simulink model "arducopter"  (R2021a)
settings: Solver=FixedStepAuto  StartTime=0.0  StopTime=simIn.param.timeEnd  FixedStep=simIn.param.dt  RelTol=1e-3
undefined symbols (not defined in the file or in its folder): DiscIntNeverNeededParam, sim, simIn
libraries: simulink x35, slident x4, vrlib x1
(part 5 of 9)

== system arducopter/Rate Controller/PID Pitch Rate/RAT_FLTD ==
  note: See AP_Math.cpp, calc_lowpass_alpha_dt()
  note: See AC_PID.cpp, update_all()
  note: Alpha Calculation:
      | $\alpha = \frac{\mathrm{d}t}{\mathrm{d}t + 2 \pi f_{\mathrm{Cutoff}}$
  note: Digital Filter:
      | $y_n = (1 - \alpha)y_{n-1} + x \cdot \alpha$
  u : Inport
  cutoff_freq : Inport  Port=2
  ATC input time constant : Constant  Value=simIn.param.dt
  Add : Sum
  Calculate Alpha : Product  Inputs=*/
  Compare To Zero : simulink/Logic and Bit Operations/Compare To Zero  relop=<=  OutDataTypeStr=boolean
  Compare To Zero1 : simulink/Logic and Bit Operations/Compare To Zero  relop=<=  OutDataTypeStr=boolean
  Constant2 : Constant  OutDataTypeStr=single
  Constant3 : Constant  OutDataTypeStr=single
  Constant4 : Constant  OutDataTypeStr=single
  Data Type Conversion1 : DataTypeConversion  OutDataTypeStr=single
  Divide : Product  Inputs=*/
  Gain : Gain  Gain=2*pi
  IC : InitialCondition  Value=simIn.init.PIDP.DerFilt
  Logical Operator : Logic  Operator=OR  AllPortsSameDT=off  OutDataTypeStr=boolean
  Product : Product
  Product1 : Product
  Subtract1 : Sum  Inputs=+-
  Sum : Sum  Inputs=++|
  Switch : Switch  Criteria=u2 > Threshold
  Unit Delay : UnitDelay  SampleTime=-1  HasFrameUpgradeWarning=on
  y : Outport
  wires:
  IC/1 -> y/1, Unit Delay/1
  Sum/1 -> IC/1
  Constant4/1 -> Switch/1
  Logical Operator/1 -> Switch/2
  Compare To Zero1/1 -> Logical Operator/2
  Compare To Zero/1 -> Logical Operator/1
  [cutoff_freq] -> Compare To Zero1/1
  [dt] -> Compare To Zero/1
  [cutoff_freq] -> Gain/1
  ATC input time constant/1 -> Data Type Conversion1/1
  Switch/1 -> [alpha]
  Product/1 -> Sum/1
  Constant3/1 -> Divide/1
  Divide/1 -> Add/2
  u/1 -> Product/2
  cutoff_freq/1 -> [cutoff_freq]
  Gain/1 -> Divide/2
  [dt] -> Calculate Alpha/1, Add/1
  Add/1 -> Calculate Alpha/2
  Calculate Alpha/1 -> Switch/3
  [alpha] -> Product/1
  Constant2/1 -> Subtract1/1
  [alpha] -> Subtract1/2
  Subtract1/1 -> Product1/1
  Unit Delay/1 -> Product1/2
  Product1/1 -> Sum/2
  Data Type Conversion1/1 -> [dt]

== system arducopter/Rate Controller/PID Pitch Rate/RAT_FLTE ==
  note: See AP_Math.cpp, calc_lowpass_alpha_dt()
  note: See AC_PID.cpp, update_all()
  note: Alpha Calculation:
      | $\alpha = \frac{\mathrm{d}t}{\mathrm{d}t + 2 \pi f_{\mathrm{Cutoff}}$
  note: Digital Filter:
      | $y_n = (1 - \alpha)y_{n-1} + x \cdot \alpha$
  u : Inport
  cutoff_freq : Inport  Port=2
  ATC input time constant : Constant  Value=simIn.param.dt
  Add : Sum
  Calculate Alpha : Product  Inputs=*/
  Compare To Zero : simulink/Logic and Bit Operations/Compare To Zero  relop=<=  OutDataTypeStr=boolean
  Compare To Zero1 : simulink/Logic and Bit Operations/Compare To Zero  relop=<=  OutDataTypeStr=boolean
  Constant2 : Constant  OutDataTypeStr=single
  Constant3 : Constant  OutDataTypeStr=single
  Constant4 : Constant  OutDataTypeStr=single
  Data Type Conversion1 : DataTypeConversion  OutDataTypeStr=single
  Divide : Product  Inputs=*/
  Gain : Gain  Gain=2*pi
  IC : InitialCondition  Value=simIn.init.PIDP.ErrFilt
  Logical Operator : Logic  Operator=OR  AllPortsSameDT=off  OutDataTypeStr=boolean
  Product : Product
  Product1 : Product
  Subtract1 : Sum  Inputs=+-
  Sum : Sum  Inputs=++|  OutDataTypeStr=single
  Switch : Switch  Criteria=u2 > Threshold
  Unit Delay : UnitDelay  SampleTime=-1  HasFrameUpgradeWarning=on
  y : Outport
  wires:
  IC/1 -> y/1, Unit Delay/1
  Sum/1 -> IC/1
  Constant4/1 -> Switch/1
  Logical Operator/1 -> Switch/2
  Compare To Zero1/1 -> Logical Operator/2
  Compare To Zero/1 -> Logical Operator/1
  [cutoff_freq] -> Compare To Zero1/1
  [dt] -> Compare To Zero/1
  [cutoff_freq] -> Gain/1
  ATC input time constant/1 -> Data Type Conversion1/1
  Switch/1 -> [alpha]
  Product/1 -> Sum/1
  Constant3/1 -> Divide/1
  Divide/1 -> Add/2
  u/1 -> Product/2
  cutoff_freq/1 -> [cutoff_freq]
  Gain/1 -> Divide/2
  [dt] -> Calculate Alpha/1, Add/1
  Add/1 -> Calculate Alpha/2
  Calculate Alpha/1 -> Switch/3
  [alpha] -> Product/1
  Constant2/1 -> Subtract1/1
  [alpha] -> Subtract1/2
  Subtract1/1 -> Product1/1
  Unit Delay/1 -> Product1/2
  Product1/1 -> Sum/2
  Data Type Conversion1/1 -> [dt]

== system arducopter/Rate Controller/PID Pitch Rate/RAT_FLTT ==
  note: Digital Filter:
      | $y_n = (1 - \alpha)y_{n-1} + x \cdot \alpha$
  note: Alpha Calculation:
      | $\alpha = \frac{\mathrm{d}t}{\mathrm{d}t + 2 \pi f_{\mathrm{Cutoff}}$
  note: See AC_PID.cpp, update_all()
  note: See AP_Math.cpp, calc_lowpass_alpha_dt()
  u : Inport
  cutoff_freq : Inport  Port=2
  ATC input time constant : Constant  Value=simIn.param.dt
  Add : Sum
  Calculate Alpha : Product  Inputs=*/
  Compare To Zero : simulink/Logic and Bit Operations/Compare To Zero  relop=<=  OutDataTypeStr=boolean
  Compare To Zero1 : simulink/Logic and Bit Operations/Compare To Zero  relop=<=  OutDataTypeStr=boolean
  Constant2 : Constant  OutDataTypeStr=single
  Constant3 : Constant  OutDataTypeStr=single
  Constant4 : Constant  OutDataTypeStr=single
  Data Type Conversion1 : DataTypeConversion  OutDataTypeStr=single
  Divide : Product  Inputs=*/
  Gain : Gain  Gain=2*pi
  IC : InitialCondition  Value=simIn.init.PIDP.TarFilt
  Logical Operator : Logic  Operator=OR  AllPortsSameDT=off  OutDataTypeStr=boolean
  Product : Product
  Product1 : Product
  Subtract1 : Sum  Inputs=+-
  Sum : Sum  Inputs=++|
  Switch : Switch  Criteria=u2 > Threshold
  Unit Delay : UnitDelay  SampleTime=-1  HasFrameUpgradeWarning=on
  y : Outport
  wires:
  IC/1 -> Unit Delay/1, y/1
  Unit Delay/1 -> Product1/2
  Sum/1 -> IC/1
  Product1/1 -> Sum/2
  Subtract1/1 -> Product1/1
  [alpha] -> Subtract1/2
  Constant2/1 -> Subtract1/1
  [alpha] -> Product/1
  Calculate Alpha/1 -> Switch/3
  Add/1 -> Calculate Alpha/2
  [dt] -> Add/1, Calculate Alpha/1
  Gain/1 -> Divide/2
  cutoff_freq/1 -> [cutoff_freq]
  u/1 -> Product/2
  Divide/1 -> Add/2
  Constant3/1 -> Divide/1
  Product/1 -> Sum/1
  Switch/1 -> [alpha]
  ATC input time constant/1 -> Data Type Conversion1/1
  [cutoff_freq] -> Gain/1
  [dt] -> Compare To Zero/1
  [cutoff_freq] -> Compare To Zero1/1
  Compare To Zero/1 -> Logical Operator/1
  Compare To Zero1/1 -> Logical Operator/2
  Logical Operator/1 -> Switch/2
  Constant4/1 -> Switch/1
  Data Type Conversion1/1 -> [dt]

== system arducopter/Rate Controller/PID Pitch Rate/Slew Limiter ==
  note: Data Store Memory Elements: Global variables of subsystem
  note: Slew Limiter
      |
      | Calculates the slew limit modifiert Dmod for the P and D part of the controller. The calculation of Dmod is taken from SlewLimiter::modifier() in SlewLimiter.cpp.
  p_out : Inport
  sr_max : Inport  Port=2
  sr_tau : Inport  Port=3
  sr_flt_f : Inport  Port=4
  clock : Inport  Port=5
  d_out : Inport  Port=6
  ATC sample time1 : Constant  Value=simIn.param.dt
  Calculate Dmod1 : MATLAB Function  TreatAsAtomicUnit=on  SystemSampleTime=0.0025
  Constant7 : Constant  Value=simIn.param.LOOP_RATE
  Data Store Memory : DataStoreMemory  DataStoreName=pos_event_stored  ReadBeforeWriteMsg=warning  WriteAfterWriteMsg=warning  WriteAfterReadMsg=warning  InitialValue=false  ShowAdditionalParam=off  OutDataTypeStr=boolean
  Data Store Memory1 : DataStoreMemory  DataStoreName=neg_event_stored  ReadBeforeWriteMsg=warning  WriteAfterWriteMsg=warning  WriteAfterReadMsg=warning  InitialValue=false  ShowAdditionalParam=off  OutDataTypeStr=boolean
  Data Store Memory10 : DataStoreMemory  DataStoreName=modifier_slew_rate  ReadBeforeWriteMsg=warning  WriteAfterWriteMsg=warning  WriteAfterReadMsg=warning  InitialValue=simIn.init.PIDP.SrOut  ShowAdditionalParam=off  OutDataTypeStr=single
  Data Store Memory11 : DataStoreMemory  DataStoreName=output_slew_rate  ReadBeforeWriteMsg=warning  WriteAfterWriteMsg=warning  WriteAfterReadMsg=warning  InitialValue=simIn.init.PIDP.SrOut  ShowAdditionalParam=off  OutDataTypeStr=single
  Data Store Memory2 : DataStoreMemory  DataStoreName=pos_event_idx  ReadBeforeWriteMsg=warning  WriteAfterWriteMsg=warning  WriteAfterReadMsg=warning  InitialValue=1  ShowAdditionalParam=off  OutDataTypeStr=int8
  Data Store Memory3 : DataStoreMemory  DataStoreName=neg_event_idx  ReadBeforeWriteMsg=warning  WriteAfterWriteMsg=warning  WriteAfterReadMsg=warning  InitialValue=1  ShowAdditionalParam=off  OutDataTypeStr=int8
  Data Store Memory4 : DataStoreMemory  DataStoreName=pos_event_ms  ReadBeforeWriteMsg=warning  WriteAfterWriteMsg=warning  WriteAfterReadMsg=warning  InitialValue=[0 0]  ShowAdditionalParam=off  OutDataTypeStr=uint32  Dimensions=2
  Data Store Memory5 : DataStoreMemory  DataStoreName=neg_event_ms  ReadBeforeWriteMsg=warning  WriteAfterWriteMsg=warning  WriteAfterReadMsg=warning  InitialValue=[0 0]  ShowAdditionalParam=off  OutDataTypeStr=uint32  Dimensions=2
  Data Store Memory6 : DataStoreMemory  DataStoreName=max_pos_slew_rate  ReadBeforeWriteMsg=warning  WriteAfterWriteMsg=warning  WriteAfterReadMsg=warning  ShowAdditionalParam=off  OutDataTypeStr=single
  Data Store Memory7 : DataStoreMemory  DataStoreName=max_pos_slew_event_ms  ReadBeforeWriteMsg=warning  WriteAfterWriteMsg=warning  WriteAfterReadMsg=warning  ShowAdditionalParam=off  OutDataTypeStr=uint32
  Data Store Memory8 : DataStoreMemory  DataStoreName=max_neg_slew_rate  ReadBeforeWriteMsg=warning  WriteAfterWriteMsg=warning  WriteAfterReadMsg=warning  ShowAdditionalParam=off  OutDataTypeStr=single
  Data Store Memory9 : DataStoreMemory  DataStoreName=max_neg_slew_event_ms  ReadBeforeWriteMsg=warning  WriteAfterWriteMsg=warning  WriteAfterReadMsg=warning  ShowAdditionalParam=off  OutDataTypeStr=uint32
  Data Store Read : DataStoreRead  DataStoreName=modifier_slew_rate  DataStoreElements=modifier_slew_rate  IndexOptions=Index vector (dialog)  Indices=1  OutputSizes=1
  Data Store Read1 : DataStoreRead  DataStoreName=output_slew_rate  DataStoreElements=output_slew_rate  IndexOptions=Index vector (dialog)  Indices=1  OutputSizes=1
  Data Type Conversion1 : DataTypeConversion  OutDataTypeStr=single
  IC : InitialCondition  Value=2*simIn.init.PIDP.SrOut
  Lowpass Filter1 : MATLAB Function  TreatAsAtomicUnit=on
  Subsystem : Subsystem
  Terminator : Terminator
  Terminator1 : Terminator
  Unit Delay1 : UnitDelay  SampleTime=-1  HasFrameUpgradeWarning=on
  Dmod : Outport
  wires:
  Constant7/1 -> Lowpass Filter1/3(loop_rate)
  sr_flt_f/1 -> Lowpass Filter1/2(cutoff_freq)
  Lowpass Filter1/1(out) -> IC/1  "pitchRateSrFilt"
  Unit Delay1/1 -> Lowpass Filter1/4(out_last)
  Calculate Dmod1/1(Dmod) -> Dmod/1  "pitchRateDmod"
  sr_max/1 -> Calculate Dmod1/2(sr_max)
  sr_tau/1 -> Calculate Dmod1/3(sr_tau)
  ATC sample time1/1 -> Data Type Conversion1/1
  Data Store Read/1 -> Terminator/1  "pitchRateSrMod"
  Data Store Read1/1 -> Terminator1/1  "pitchRateSrOut"
  p_out/1 -> Subsystem/1(p_out)
  d_out/1 -> Subsystem/2(d_out)
  Subsystem/1(sr_raw) -> Lowpass Filter1/1(in)  "pitchRateSrRaw"
  Data Type Conversion1/1 -> Calculate Dmod1/4(dt)
  IC/1 -> Calculate Dmod1/1(slew_rate), Unit Delay1/1
  clock/1 -> Calculate Dmod1/5(time)

== system arducopter/Rate Controller/PID Roll Rate/Calc Derivative ==
  e : Inport
  ATC input time constant : Constant  Value=simIn.param.dt
  Data Type Conversion : DataTypeConversion  OutDataTypeStr=single
  Divide : Product  Inputs=*/
  Sum : Sum  Inputs=|+-
  Unit Delay : UnitDelay  SampleTime=-1  HasFrameUpgradeWarning=on
  derivative : Outport
  wires:
  e/1 -> Sum/1, Unit Delay/1
  Unit Delay/1 -> Sum/2
  Sum/1 -> Divide/1
  ATC input time constant/1 -> Data Type Conversion/1
  Divide/1 -> derivative/1
  Data Type Conversion/1 -> Divide/2

== system arducopter/Rate Controller/PID Roll Rate/I ==
  note: Integrator, see AC_PID::update_i()
  e : Inport
  limit_flg : Inport  Port=2
  ki : Inport  Port=3
  i_max : Inport  Port=4
  Constant1 : Constant  Value=simIn.param.dt
  Data Type Conversion : DataTypeConversion  OutDataTypeStr=single
  IC1 : InitialCondition  Value=simIn.init.PIDR.I
  Integrator : MATLAB Function  TreatAsAtomicUnit=on
  Unit Delay1 : UnitDelay  SampleTime=-1  HasFrameUpgradeWarning=on
  integrator : Outport
  wires:
  [integrator_out] -> integrator/1
  Constant1/1 -> Data Type Conversion/1
  limit_flg/1 -> Integrator/3(limit_flg)
  [integrator_out] -> Unit Delay1/1
  IC1/1 -> [integrator_out]
  Unit Delay1/1 -> Integrator/2(integrator)
  ki/1 -> Integrator/4(ki)
  i_max/1 -> Integrator/5(i_max)
  e/1 -> Integrator/1(error)
  Integrator/1(integrator_out) -> IC1/1
  Data Type Conversion/1 -> Integrator/6(dt)

== system arducopter/Rate Controller/PID Roll Rate/RAT_FLTD ==
  note: Digital Filter:
      | $y_n = (1 - \alpha)y_{n-1} + x \cdot \alpha$
  note: Alpha Calculation:
      | $\alpha = \frac{\mathrm{d}t}{\mathrm{d}t + 2 \pi T_{\mathrm{Cutoff}}$
  note: See AC_PID.cpp, update_all()
  note: See AP_Math.cpp, calc_lowpass_alpha_dt()
  u : Inport
  cutoff_freq : Inport  Port=2
  ATC input time constant : Constant  Value=simIn.param.dt
  Add : Sum
  Calculate Alpha : Product  Inputs=*/
  Compare To Zero : simulink/Logic and Bit Operations/Compare To Zero  relop=<=  OutDataTypeStr=boolean
  Compare To Zero1 : simulink/Logic and Bit Operations/Compare To Zero  relop=<=  OutDataTypeStr=boolean
  Constant : Constant  Commented=on
  Constant1 : Constant  Commented=on
  Constant2 : Constant  OutDataTypeStr=single
  Constant3 : Constant  OutDataTypeStr=single
  Constant4 : Constant  OutDataTypeStr=single
  Data Type Conversion : DataTypeConversion  OutDataTypeStr=single
  Discrete Filter : DiscreteFilter  Commented=on  NumeratorSource=Input port  DenominatorSource=Input port  a0EqualsOne=on
      settings: InputPortMap=u0,p1,p3
  Divide : Product  Inputs=*/
  From : From  Commented=on  GotoTag=alpha
  From1 : From  Commented=on  GotoTag=alpha
  Gain : Gain  Gain=2*pi
  Gain1 : Gain  Commented=on  Gain=-1
  IC : InitialCondition  Value=simIn.init.PIDR.DerFilt
  Logical Operator : Logic  Operator=OR  AllPortsSameDT=off  OutDataTypeStr=boolean
  Product : Product
  Product1 : Product
  Subtract : Sum  Commented=on  Inputs=+-
  Subtract1 : Sum  Inputs=+-
  Sum : Sum  Inputs=++|  AccumDataTypeStr=single
  Switch : Switch  Criteria=u2 > Threshold
  Unit Delay : UnitDelay  SampleTime=-1  HasFrameUpgradeWarning=on
  Vector Concatenate : Concatenate  Commented=on
  degree2radian1 : Gain  Commented=on  Gain=pi/180
  y : Outport
  wires:
  Product1/1 -> Sum/2
  Unit Delay/1 -> Product1/2
  Subtract1/1 -> Product1/1
  [alpha] -> Subtract1/2
  Constant2/1 -> Subtract1/1
  [alpha] -> Product/1
  Vector Concatenate/1 -> Discrete Filter/3
  Constant1/1 -> Vector Concatenate/1
  Gain1/1 -> Vector Concatenate/2
  Subtract/1 -> Gain1/1
  Constant/1 -> Subtract/1
  From1/1 -> Subtract/2
  From/1 -> Discrete Filter/2
  Calculate Alpha/1 -> Switch/3
  Add/1 -> Calculate Alpha/2
  [dt] -> Add/1, Calculate Alpha/1
  Gain/1 -> Divide/2
  cutoff_freq/1 -> [cutoff_freq]
  Discrete Filter/1 -> degree2radian1/1
  u/1 -> Product/2
  Divide/1 -> Add/2
  Constant3/1 -> Divide/1
  Product/1 -> Sum/1
  Switch/1 -> [alpha]
  ATC input time constant/1 -> Data Type Conversion/1
  [cutoff_freq] -> Gain/1
  [dt] -> Compare To Zero/1
  [cutoff_freq] -> Compare To Zero1/1
  Compare To Zero/1 -> Logical Operator/1
  Compare To Zero1/1 -> Logical Operator/2
  Logical Operator/1 -> Switch/2
  Constant4/1 -> Switch/1
  Sum/1 -> IC/1
  IC/1 -> Unit Delay/1, y/1
  Data Type Conversion/1 -> [dt]

== system arducopter/Rate Controller/PID Roll Rate/RAT_FLTE ==
  note: Digital Filter:
      | $y_n = (1 - \alpha)y_{n-1} + x \cdot \alpha$
  note: Alpha Calculation:
      | $\alpha = \frac{\mathrm{d}t}{\mathrm{d}t + 2 \pi f_{\mathrm{Cutoff}}$
  note: See AC_PID.cpp, update_all()
  note: See AP_Math.cpp, calc_lowpass_alpha_dt()
  u : Inport
  cutoff_freq : Inport  Port=2
  ATC input time constant : Constant  Value=simIn.param.dt
  Add : Sum
  Calculate Alpha : Product  Inputs=*/
  Compare To Zero : simulink/Logic and Bit Operations/Compare To Zero  relop=<=  OutDataTypeStr=boolean
  Compare To Zero1 : simulink/Logic and Bit Operations/Compare To Zero  relop=<=  OutDataTypeStr=boolean
  Constant2 : Constant  OutDataTypeStr=single
  Constant3 : Constant  OutDataTypeStr=single
  Constant4 : Constant  OutDataTypeStr=single
  Data Type Conversion : DataTypeConversion  OutDataTypeStr=single
  Divide : Product  Inputs=*/
  Gain : Gain  Gain=2*pi
  IC : InitialCondition  Value=simIn.init.PIDR.ErrFilt
  Logical Operator : Logic  Operator=OR  AllPortsSameDT=off  OutDataTypeStr=boolean
  Product : Product
  Product1 : Product
  Subtract1 : Sum  Inputs=+-
  Sum : Sum  Inputs=++|  OutDataTypeStr=single
  Switch : Switch  Criteria=u2 > Threshold
  Unit Delay : UnitDelay  SampleTime=-1  HasFrameUpgradeWarning=on
  y : Outport
  wires:
  Product1/1 -> Sum/2
  Unit Delay/1 -> Product1/2
  Subtract1/1 -> Product1/1
  [alpha] -> Subtract1/2
  Constant2/1 -> Subtract1/1
  [alpha] -> Product/1
  Calculate Alpha/1 -> Switch/3
  Add/1 -> Calculate Alpha/2
  [dt] -> Add/1, Calculate Alpha/1
  Gain/1 -> Divide/2
  cutoff_freq/1 -> [cutoff_freq]
  u/1 -> Product/2
  Divide/1 -> Add/2
  Constant3/1 -> Divide/1
  Product/1 -> Sum/1
  Switch/1 -> [alpha]
  ATC input time constant/1 -> Data Type Conversion/1
  [cutoff_freq] -> Gain/1
  [dt] -> Compare To Zero/1
  [cutoff_freq] -> Compare To Zero1/1
  Compare To Zero/1 -> Logical Operator/1
  Compare To Zero1/1 -> Logical Operator/2
  Logical Operator/1 -> Switch/2
  Constant4/1 -> Switch/1
  Sum/1 -> IC/1
  IC/1 -> Unit Delay/1, y/1
  Data Type Conversion/1 -> [dt]

== system arducopter/Rate Controller/PID Roll Rate/RAT_FLTT ==
  note: See AP_Math.cpp, calc_lowpass_alpha_dt()
  note: See AC_PID.cpp, update_all()
  note: Alpha Calculation:
      | $\alpha = \frac{\mathrm{d}t}{\mathrm{d}t + 2 \pi f_{\mathrm{Cutoff}}$
  note: Digital Filter:
      | $y_n = (1 - \alpha)y_{n-1} + x \cdot \alpha$
  u : Inport
  cutoff_freq : Inport  Port=2
  ATC input time constant : Constant  Value=simIn.param.dt
  Add : Sum
  Calculate Alpha : Product  Inputs=*/
  Compare To Zero : simulink/Logic and Bit Operations/Compare To Zero  relop=<=  OutDataTypeStr=boolean
  Compare To Zero1 : simulink/Logic and Bit Operations/Compare To Zero  relop=<=  OutDataTypeStr=boolean
  Constant2 : Constant  OutDataTypeStr=single
  Constant3 : Constant  OutDataTypeStr=single
  Constant4 : Constant  OutDataTypeStr=single
  Data Type Conversion : DataTypeConversion  OutDataTypeStr=single
  Divide : Product  Inputs=*/
  Gain : Gain  Gain=2*pi
  IC : InitialCondition  Value=simIn.init.PIDR.TarFilt
  Logical Operator : Logic  Operator=OR  AllPortsSameDT=off  OutDataTypeStr=boolean
  Product : Product
  Product1 : Product
  Subtract1 : Sum  Inputs=+-
  Sum : Sum  Inputs=++|
  Switch : Switch  Criteria=u2 > Threshold
  Unit Delay : UnitDelay  SampleTime=-1  HasFrameUpgradeWarning=on
  y : Outport
  wires:
  Constant4/1 -> Switch/1
  Logical Operator/1 -> Switch/2
  Compare To Zero1/1 -> Logical Operator/2
  Compare To Zero/1 -> Logical Operator/1
  [cutoff_freq] -> Compare To Zero1/1
  [dt] -> Compare To Zero/1
  [cutoff_freq] -> Gain/1
  ATC input time constant/1 -> Data Type Conversion/1
  Switch/1 -> [alpha]
  Product/1 -> Sum/1
  Constant3/1 -> Divide/1
  Divide/1 -> Add/2
  u/1 -> Product/2
  cutoff_freq/1 -> [cutoff_freq]
  Gain/1 -> Divide/2
  [dt] -> Calculate Alpha/1, Add/1
  Add/1 -> Calculate Alpha/2
  Calculate Alpha/1 -> Switch/3
  [alpha] -> Product/1
  Constant2/1 -> Subtract1/1
  [alpha] -> Subtract1/2
  Subtract1/1 -> Product1/1
  Product1/1 -> Sum/2
  Sum/1 -> IC/1
  Unit Delay/1 -> Product1/2
  IC/1 -> y/1, Unit Delay/1
  Data Type Conversion/1 -> [dt]

== system arducopter/Rate Controller/PID Roll Rate/Slew Limiter ==
  note: Data Store Memory Elements: Global variables of subsystem
  note: Slew Limiter
      |
      | Calculates the slew limit modifiert Dmod for the P and D part of the controller. The calculation of Dmod is taken from SlewLimiter::modifier() in SlewLimiter.cpp.
  p_out : Inport
  sr_max : Inport  Port=2
  sr_tau : Inport  Port=3
  sr_flt_f : Inport  Port=4
  clock : Inport  Port=5
  d_out : Inport  Port=6
  Calculate Dmod : MATLAB Function  TreatAsAtomicUnit=on  SystemSampleTime=0.0025
  Constant7 : Constant  Value=simIn.param.LOOP_RATE
  Data Store Memory : DataStoreMemory  DataStoreName=pos_event_stored  ReadBeforeWriteMsg=warning  WriteAfterWriteMsg=warning  WriteAfterReadMsg=warning  InitialValue=false  ShowAdditionalParam=off  OutDataTypeStr=boolean
  Data Store Memory1 : DataStoreMemory  DataStoreName=neg_event_stored  ReadBeforeWriteMsg=warning  WriteAfterWriteMsg=warning  WriteAfterReadMsg=warning  InitialValue=false  ShowAdditionalParam=off  OutDataTypeStr=boolean
  Data Store Memory10 : DataStoreMemory  DataStoreName=modifier_slew_rate  ReadBeforeWriteMsg=warning  WriteAfterWriteMsg=warning  WriteAfterReadMsg=warning  InitialValue=simIn.init.PIDR.SROut  ShowAdditionalParam=off  OutDataTypeStr=single
  Data Store Memory11 : DataStoreMemory  DataStoreName=output_slew_rate  ReadBeforeWriteMsg=warning  WriteAfterWriteMsg=warning  WriteAfterReadMsg=warning  InitialValue=simIn.init.PIDR.SROut  ShowAdditionalParam=off  OutDataTypeStr=single
  Data Store Memory2 : DataStoreMemory  DataStoreName=pos_event_idx  ReadBeforeWriteMsg=warning  WriteAfterWriteMsg=warning  WriteAfterReadMsg=warning  InitialValue=1  ShowAdditionalParam=off  OutDataTypeStr=int8
  Data Store Memory3 : DataStoreMemory  DataStoreName=neg_event_idx  ReadBeforeWriteMsg=warning  WriteAfterWriteMsg=warning  WriteAfterReadMsg=warning  InitialValue=1  ShowAdditionalParam=off  OutDataTypeStr=int8
  Data Store Memory4 : DataStoreMemory  DataStoreName=pos_event_ms  ReadBeforeWriteMsg=warning  WriteAfterWriteMsg=warning  WriteAfterReadMsg=warning  InitialValue=[0 0]  ShowAdditionalParam=off  OutDataTypeStr=uint32  Dimensions=2
  Data Store Memory5 : DataStoreMemory  DataStoreName=neg_event_ms  ReadBeforeWriteMsg=warning  WriteAfterWriteMsg=warning  WriteAfterReadMsg=warning  InitialValue=[0 0]  ShowAdditionalParam=off  OutDataTypeStr=uint32  Dimensions=2
  Data Store Memory6 : DataStoreMemory  DataStoreName=max_pos_slew_rate  ReadBeforeWriteMsg=warning  WriteAfterWriteMsg=warning  WriteAfterReadMsg=warning  ShowAdditionalParam=off  OutDataTypeStr=single
  Data Store Memory7 : DataStoreMemory  DataStoreName=max_pos_slew_event_ms  ReadBeforeWriteMsg=warning  WriteAfterWriteMsg=warning  WriteAfterReadMsg=warning  ShowAdditionalParam=off  OutDataTypeStr=uint32
  Data Store Memory8 : DataStoreMemory  DataStoreName=max_neg_slew_rate  ReadBeforeWriteMsg=warning  WriteAfterWriteMsg=warning  WriteAfterReadMsg=warning  ShowAdditionalParam=off  OutDataTypeStr=single
  Data Store Memory9 : DataStoreMemory  DataStoreName=max_neg_slew_event_ms  ReadBeforeWriteMsg=warning  WriteAfterWriteMsg=warning  WriteAfterReadMsg=warning  ShowAdditionalParam=off  OutDataTypeStr=uint32
  Data Store Read : DataStoreRead  DataStoreName=modifier_slew_rate  DataStoreElements=modifier_slew_rate  IndexOptions=Index vector (dialog)  Indices=1  OutputSizes=1
  Data Store Read1 : DataStoreRead  DataStoreName=output_slew_rate  DataStoreElements=output_slew_rate  IndexOptions=Index vector (dialog)  Indices=1  OutputSizes=1
  Data Type Conversion1 : DataTypeConversion  OutDataTypeStr=single
  IC : InitialCondition  Value=2*simIn.init.PIDR.SROut
  Lowpass Filter : MATLAB Function  TreatAsAtomicUnit=on
  Sample time : Constant  Value=simIn.param.dt
  Subsystem : Subsystem
  Terminator : Terminator
  Terminator1 : Terminator
  Unit Delay1 : UnitDelay  SampleTime=-1  HasFrameUpgradeWarning=on
  Dmod : Outport
  wires:
  Constant7/1 -> Lowpass Filter/3(loop_rate)
  sr_flt_f/1 -> Lowpass Filter/2(cutoff_freq)
  Lowpass Filter/1(out) -> IC/1  "rollRateSrFilt"
  Unit Delay1/1 -> Lowpass Filter/4(out_last)
  Calculate Dmod/1(Dmod) -> Dmod/1  "rollRateDmod"
  sr_max/1 -> Calculate Dmod/2(sr_max)
  sr_tau/1 -> Calculate Dmod/3(sr_tau)
  Sample time/1 -> Data Type Conversion1/1
  Data Store Read/1 -> Terminator/1  "rollRateSrModifier"
  Data Store Read1/1 -> Terminator1/1  "rollRateSrOut"
  p_out/1 -> Subsystem/1(p_out)
  d_out/1 -> Subsystem/2(d_out)
  Subsystem/1(sr_raw) -> Lowpass Filter/1(in)  "rollRateSrRaw"
  Data Type Conversion1/1 -> Calculate Dmod/4(dt)
  IC/1 -> Calculate Dmod/1(slew_rate), Unit Delay1/1
  clock/1 -> Calculate Dmod/5(time)

== system arducopter/Rate Controller/PID Yaw Rate/Calc Derivative ==
  e : Inport
  ATC input time constant : Constant  Value=simIn.param.dt
  Divide : Product  Inputs=*/
  Sum : Sum  Inputs=|+-
  Unit Delay : UnitDelay  SampleTime=-1  HasFrameUpgradeWarning=on
  derivative : Outport
  wires:
  e/1 -> Sum/1, Unit Delay/1
  Unit Delay/1 -> Sum/2
  Sum/1 -> Divide/1
  ATC input time constant/1 -> Divide/2
  Divide/1 -> derivative/1

== system arducopter/Rate Controller/PID Yaw Rate/I ==
  note: Integrator, see AC_PID::update_i()
  e : Inport
  limit_flg : Inport  Port=2
  ki : Inport  Port=3
  i_max : Inport  Port=4
  Constant1 : Constant  Value=simIn.param.dt
  Data Type Conversion1 : DataTypeConversion  OutDataTypeStr=single
  IC1 : InitialCondition  Value=simIn.init.PIDY.I
  Integrator : MATLAB Function  TreatAsAtomicUnit=on
  Unit Delay1 : UnitDelay  InitialCondition=single(0)  SampleTime=-1  HasFrameUpgradeWarning=on
  integrator : Outport
  wires:
  e/1 -> Integrator/1(error)
  Integrator/1(integrator_out) -> IC1/1
  [integrator_out] -> integrator/1
  Constant1/1 -> Data Type Conversion1/1
  limit_flg/1 -> Integrator/3(limit_flg)
  [integrator_out] -> Unit Delay1/1
  IC1/1 -> [integrator_out]
  Unit Delay1/1 -> Integrator/2(integrator)
  ki/1 -> Integrator/4(ki)
  i_max/1 -> Integrator/5(i_max)
  Data Type Conversion1/1 -> Integrator/6(dt)

== system arducopter/Rate Controller/PID Yaw Rate/RAT_FLTD ==
  note: Digital Filter:
      | $y_n = (1 - \alpha)y_{n-1} + x \cdot \alpha$
  note: Alpha Calculation:
      | $\alpha = \frac{\mathrm{d}t}{\mathrm{d}t + 2 \pi f_{\mathrm{Cutoff}}$
  note: See AC_PID.cpp, update_all()
  note: See AP_Math.cpp, line 393.
  u : Inport
  cutoff_freq : Inport  Port=2
  ATC input time constant : Constant  Value=simIn.param.dt
  Add : Sum
  Calculate Alpha : Product  Inputs=*/
  Compare To Zero : simulink/Logic and Bit Operations/Compare To Zero  relop=<=  OutDataTypeStr=boolean
  Compare To Zero1 : simulink/Logic and Bit Operations/Compare To Zero  relop=<=  OutDataTypeStr=boolean
  Constant2 : Constant  OutDataTypeStr=single
  Constant3 : Constant  OutDataTypeStr=single
  Constant4 : Constant  OutDataTypeStr=single
  Data Type Conversion1 : DataTypeConversion  OutDataTypeStr=single
  Divide : Product  Inputs=*/
  Gain : Gain  Gain=2*pi
  IC : InitialCondition  Value=simIn.init.PIDY.DerFilt
  Logical Operator : Logic  Operator=OR  AllPortsSameDT=off  OutDataTypeStr=boolean
  Product : Product
  Product1 : Product
  Subtract1 : Sum  Inputs=+-
  Sum : Sum  Inputs=++|  OutDataTypeStr=single
  Switch : Switch  Criteria=u2 > Threshold
  Unit Delay : UnitDelay  SampleTime=-1  HasFrameUpgradeWarning=on
  y : Outport
  wires:
  Product1/1 -> Sum/2
  Unit Delay/1 -> Product1/2
  Subtract1/1 -> Product1/1
  [alpha] -> Subtract1/2
  Constant2/1 -> Subtract1/1
  [alpha] -> Product/1
  Calculate Alpha/1 -> Switch/3
  Add/1 -> Calculate Alpha/2
  [dt] -> Add/1, Calculate Alpha/1
  Gain/1 -> Divide/2
  cutoff_freq/1 -> [cutoff_freq]
  u/1 -> Product/2
  Divide/1 -> Add/2
  Constant3/1 -> Divide/1
  Product/1 -> Sum/1
  Switch/1 -> [alpha]
  ATC input time constant/1 -> Data Type Conversion1/1
  [cutoff_freq] -> Gain/1
  [dt] -> Compare To Zero/1
  [cutoff_freq] -> Compare To Zero1/1
  Compare To Zero/1 -> Logical Operator/1
  Compare To Zero1/1 -> Logical Operator/2
  Logical Operator/1 -> Switch/2
  Constant4/1 -> Switch/1
  Sum/1 -> IC/1
  IC/1 -> Unit Delay/1, y/1
  Data Type Conversion1/1 -> [dt]

== system arducopter/Rate Controller/PID Yaw Rate/RAT_FLTE ==
  note: Digital Filter:
      | $y_n = (1 - \alpha)y_{n-1} + x \cdot \alpha$
  note: Alpha Calculation:
      | $\alpha = \frac{\mathrm{d}t}{\mathrm{d}t + 2 \pi f_{\mathrm{Cutoff}}$
  note: See AC_PID.cpp, update_all()
  note: See AP_Math.cpp, line 393.
  u : Inport
  cutoff_freq : Inport  Port=2
  ATC input time constant : Constant  Value=simIn.param.dt
  Add : Sum
  Calculate Alpha : Product  Inputs=*/
  Compare To Zero : simulink/Logic and Bit Operations/Compare To Zero  relop=<=  OutDataTypeStr=boolean
  Compare To Zero1 : simulink/Logic and Bit Operations/Compare To Zero  relop=<=  OutDataTypeStr=boolean
  Constant : Constant  Commented=on
  Constant1 : Constant  Commented=on
  Constant2 : Constant  OutDataTypeStr=single
  Constant3 : Constant  OutDataTypeStr=single
  Constant4 : Constant  OutDataTypeStr=single
  Data Type Conversion1 : DataTypeConversion  OutDataTypeStr=single
  Discrete Filter : DiscreteFilter  Commented=on  NumeratorSource=Input port  DenominatorSource=Input port  a0EqualsOne=on
      settings: InputPortMap=u0,p1,p3
  Divide : Product  Inputs=*/
  From : From  Commented=on  GotoTag=alpha
  From1 : From  Commented=on  GotoTag=alpha
  Gain : Gain  Gain=2*pi
  Gain1 : Gain  Commented=on  Gain=-1
  IC : InitialCondition  Value=simIn.init.PIDY.ErrFilt
  Logical Operator : Logic  Operator=OR  AllPortsSameDT=off  OutDataTypeStr=boolean
  Product : Product
  Product1 : Product
  Subtract : Sum  Commented=on  Inputs=+-
  Subtract1 : Sum  Inputs=+-
  Sum : Sum  Inputs=++|  OutDataTypeStr=single
  Switch : Switch  Criteria=u2 > Threshold
  Unit Delay : UnitDelay  SampleTime=-1  HasFrameUpgradeWarning=on
  Vector Concatenate : Concatenate  Commented=on
  degree2radian1 : Gain  Commented=on  Gain=pi/180
  y : Outport
  wires:
  Product1/1 -> Sum/2
  Unit Delay/1 -> Product1/2
  Subtract1/1 -> Product1/1
  [alpha] -> Subtract1/2
  Constant2/1 -> Subtract1/1
  [alpha] -> Product/1
  Vector Concatenate/1 -> Discrete Filter/3
  Constant1/1 -> Vector Concatenate/1
  Gain1/1 -> Vector Concatenate/2
  Subtract/1 -> Gain1/1
  Constant/1 -> Subtract/1
  From1/1 -> Subtract/2
  From/1 -> Discrete Filter/2
  Calculate Alpha/1 -> Switch/3
  Add/1 -> Calculate Alpha/2
  [dt] -> Add/1, Calculate Alpha/1
  Gain/1 -> Divide/2
  cutoff_freq/1 -> [cutoff_freq]
  Discrete Filter/1 -> degree2radian1/1
  u/1 -> Product/2
  Divide/1 -> Add/2
  Constant3/1 -> Divide/1
  Product/1 -> Sum/1
  Switch/1 -> [alpha]
  ATC input time constant/1 -> Data Type Conversion1/1
  [cutoff_freq] -> Gain/1
  [dt] -> Compare To Zero/1
  [cutoff_freq] -> Compare To Zero1/1
  Compare To Zero/1 -> Logical Operator/1
  Compare To Zero1/1 -> Logical Operator/2
  Logical Operator/1 -> Switch/2
  Constant4/1 -> Switch/1
  Sum/1 -> IC/1
  IC/1 -> Unit Delay/1, y/1
  Data Type Conversion1/1 -> [dt]

== system arducopter/Rate Controller/PID Yaw Rate/RAT_FLTT ==
  note: See AP_Math.cpp, line 393.
  note: See AC_PID.cpp, update_all()
  note: Alpha Calculation:
      | $\alpha = \frac{\mathrm{d}t}{\mathrm{d}t + 2 \pi f_{\mathrm{Cutoff}}$
  note: Digital Filter:
      | $y_n = (1 - \alpha)y_{n-1} + x \cdot \alpha$
  u : Inport
  cutoff_freq : Inport  Port=2
  ATC input time constant : Constant  Value=simIn.param.dt
  Add : Sum
  Calculate Alpha : Product  Inputs=*/
  Compare To Zero : simulink/Logic and Bit Operations/Compare To Zero  relop=<=  OutDataTypeStr=boolean
  Compare To Zero1 : simulink/Logic and Bit Operations/Compare To Zero  relop=<=  OutDataTypeStr=boolean
  Constant : Constant  Commented=on
  Constant1 : Constant  Commented=on
  Constant2 : Constant  OutDataTypeStr=single
  Constant3 : Constant  OutDataTypeStr=single
  Constant4 : Constant  OutDataTypeStr=single
  Data Type Conversion1 : DataTypeConversion  OutDataTypeStr=single
  Discrete Filter : DiscreteFilter  Commented=on  NumeratorSource=Input port  DenominatorSource=Input port  a0EqualsOne=on
      settings: InputPortMap=u0,p1,p3
  Divide : Product  Inputs=*/
  From : From  Commented=on  GotoTag=alpha
  From1 : From  Commented=on  GotoTag=alpha
  Gain : Gain  Gain=2*pi
  Gain1 : Gain  Commented=on  Gain=-1
  IC : InitialCondition  Value=simIn.init.PIDY.TarFilt
  Logical Operator : Logic  Operator=OR  AllPortsSameDT=off  OutDataTypeStr=boolean
  Product : Product
  Product1 : Product
  Subtract : Sum  Commented=on  Inputs=+-
  Subtract1 : Sum  Inputs=+-
  Sum : Sum  Inputs=++|
  Switch : Switch  Criteria=u2 > Threshold
  Unit Delay : UnitDelay  SampleTime=-1  HasFrameUpgradeWarning=on
  Vector Concatenate : Concatenate  Commented=on
  degree2radian1 : Gain  Commented=on  Gain=pi/180
  y : Outport
  wires:
  Constant4/1 -> Switch/1
  Logical Operator/1 -> Switch/2
  Compare To Zero1/1 -> Logical Operator/2
  Compare To Zero/1 -> Logical Operator/1
  [cutoff_freq] -> Compare To Zero1/1
  [dt] -> Compare To Zero/1
  [cutoff_freq] -> Gain/1
  ATC input time constant/1 -> Data Type Conversion1/1
  Switch/1 -> [alpha]
  Product/1 -> Sum/1
  Constant3/1 -> Divide/1
  Divide/1 -> Add/2
  u/1 -> Product/2
  Discrete Filter/1 -> degree2radian1/1
  cutoff_freq/1 -> [cutoff_freq]
  Gain/1 -> Divide/2
  [dt] -> Calculate Alpha/1, Add/1
  Add/1 -> Calculate Alpha/2
  Calculate Alpha/1 -> Switch/3
  From/1 -> Discrete Filter/2
  From1/1 -> Subtract/2
  Constant/1 -> Subtract/1
  Subtract/1 -> Gain1/1
  Gain1/1 -> Vector Concatenate/2
  Constant1/1 -> Vector Concatenate/1
  Vector Concatenate/1 -> Discrete Filter/3
  [alpha] -> Product/1
  Constant2/1 -> Subtract1/1
  [alpha] -> Subtract1/2
  Subtract1/1 -> Product1/1
  Product1/1 -> Sum/2
  Sum/1 -> IC/1
  Unit Delay/1 -> Product1/2
  IC/1 -> y/1, Unit Delay/1
  Data Type Conversion1/1 -> [dt]

== system arducopter/Rate Controller/PID Yaw Rate/Slew Limiter ==
  note: Data Store Memory Elements: Global variables of subsystem
  note: Slew Limiter
      |
      | Calculates the slew limit modifiert Dmod for the P and D part of the controller. The calculation of Dmod is taken from SlewLimiter::modifier() in SlewLimiter.cpp.
  p_out : Inport
  sr_max : Inport  Port=2
  sr_tau : Inport  Port=3
  sr_flt_f : Inport  Port=4
  clock : Inport  Port=5
  d_out : Inport  Port=6
  ATC sample time1 : Constant  Value=simIn.param.dt
  Calculate Dmod : MATLAB Function  TreatAsAtomicUnit=on  SystemSampleTime=0.0025
  Constant7 : Constant  Value=simIn.param.dt
  Data Store Memory : DataStoreMemory  DataStoreName=pos_event_stored  ReadBeforeWriteMsg=warning  WriteAfterWriteMsg=warning  WriteAfterReadMsg=warning  InitialValue=false  ShowAdditionalParam=off  OutDataTypeStr=boolean
  Data Store Memory1 : DataStoreMemory  DataStoreName=neg_event_stored  ReadBeforeWriteMsg=warning  WriteAfterWriteMsg=warning  WriteAfterReadMsg=warning  InitialValue=false  ShowAdditionalParam=off  OutDataTypeStr=boolean
  Data Store Memory10 : DataStoreMemory  DataStoreName=modifier_slew_rate  ReadBeforeWriteMsg=warning  WriteAfterWriteMsg=warning  WriteAfterReadMsg=warning  InitialValue=simIn.init.PIDY.SrOut  ShowAdditionalParam=off  OutDataTypeStr=single
  Data Store Memory11 : DataStoreMemory  DataStoreName=output_slew_rate  ReadBeforeWriteMsg=warning  WriteAfterWriteMsg=warning  WriteAfterReadMsg=warning  InitialValue=simIn.init.PIDY.SrOut  ShowAdditionalParam=off  OutDataTypeStr=single
  Data Store Memory2 : DataStoreMemory  DataStoreName=pos_event_idx  ReadBeforeWriteMsg=warning  WriteAfterWriteMsg=warning  WriteAfterReadMsg=warning  InitialValue=1  ShowAdditionalParam=off  OutDataTypeStr=int8
  Data Store Memory3 : DataStoreMemory  DataStoreName=neg_event_idx  ReadBeforeWriteMsg=warning  WriteAfterWriteMsg=warning  WriteAfterReadMsg=warning  InitialValue=1  ShowAdditionalParam=off  OutDataTypeStr=int8
  Data Store Memory4 : DataStoreMemory  DataStoreName=pos_event_ms  ReadBeforeWriteMsg=warning  WriteAfterWriteMsg=warning  WriteAfterReadMsg=warning  InitialValue=[0 0]  ShowAdditionalParam=off  OutDataTypeStr=uint32  Dimensions=2
  Data Store Memory5 : DataStoreMemory  DataStoreName=neg_event_ms  ReadBeforeWriteMsg=warning  WriteAfterWriteMsg=warning  WriteAfterReadMsg=warning  InitialValue=[0 0]  ShowAdditionalParam=off  OutDataTypeStr=uint32  Dimensions=2
  Data Store Memory6 : DataStoreMemory  DataStoreName=max_pos_slew_rate  ReadBeforeWriteMsg=warning  WriteAfterWriteMsg=warning  WriteAfterReadMsg=warning  ShowAdditionalParam=off  OutDataTypeStr=single
  Data Store Memory7 : DataStoreMemory  DataStoreName=max_pos_slew_event_ms  ReadBeforeWriteMsg=warning  WriteAfterWriteMsg=warning  WriteAfterReadMsg=warning  ShowAdditionalParam=off  OutDataTypeStr=uint32
  Data Store Memory8 : DataStoreMemory  DataStoreName=max_neg_slew_rate  ReadBeforeWriteMsg=warning  WriteAfterWriteMsg=warning  WriteAfterReadMsg=warning  ShowAdditionalParam=off  OutDataTypeStr=single
  Data Store Memory9 : DataStoreMemory  DataStoreName=max_neg_slew_event_ms  ReadBeforeWriteMsg=warning  WriteAfterWriteMsg=warning  WriteAfterReadMsg=warning  ShowAdditionalParam=off  OutDataTypeStr=uint32
  Data Store Read : DataStoreRead  DataStoreName=modifier_slew_rate  DataStoreElements=modifier_slew_rate  IndexOptions=Index vector (dialog)  Indices=1  OutputSizes=1
  Data Store Read1 : DataStoreRead  DataStoreName=output_slew_rate  DataStoreElements=output_slew_rate  IndexOptions=Index vector (dialog)  Indices=1  OutputSizes=1
  Data Type Conversion1 : DataTypeConversion  OutDataTypeStr=single
  IC : InitialCondition  Value=2*simIn.init.PIDY.SrOut
  Lowpass Filter : MATLAB Function  TreatAsAtomicUnit=on
  Subsystem : Subsystem
  Terminator : Terminator
  Terminator1 : Terminator
  Unit Delay1 : UnitDelay  SampleTime=-1  HasFrameUpgradeWarning=on
  Dmod : Outport
  wires:
  Constant7/1 -> Lowpass Filter/3(loop_rate)
  sr_flt_f/1 -> Lowpass Filter/2(cutoff_freq)
  Lowpass Filter/1(out) -> IC/1  "yawRateSrFilt"
  Unit Delay1/1 -> Lowpass Filter/4(out_last)
  Calculate Dmod/1(Dmod) -> Dmod/1  "yawRateDmod"
  sr_max/1 -> Calculate Dmod/2(sr_max)
  sr_tau/1 -> Calculate Dmod/3(sr_tau)
  ATC sample time1/1 -> Data Type Conversion1/1
  Data Store Read/1 -> Terminator/1  "yawRateSrModifier"
  Data Store Read1/1 -> Terminator1/1  "yawRateSrOut"
  p_out/1 -> Subsystem/1(p_out)
  d_out/1 -> Subsystem/2(d_out)
  Subsystem/1(sr_raw) -> Lowpass Filter/1(in)  "yawRateSrRaw"
  Data Type Conversion1/1 -> Calculate Dmod/4(dt)
  IC/1 -> Unit Delay1/1, Calculate Dmod/1(slew_rate)
  clock/1 -> Calculate Dmod/5(time)

== system arducopter/Throttle/Throttle Calculations/Air density Calculation ==
  note: Calculation of the air density from the barometer signals.
      |
      | In order to determine the compensation gain, the air density ratio is calculated in this subsystem from the barometer measurement signals. This subsystem is only used for validation purposes.
      |
      | The calculations are based on the get_air_density() function in AP_Baro.cpp and the get_EAS2TAS() function (AP_Baro.cpp), which is called from there. The variable air_density_ratio for the air density ratio, which is used for the calculation of the compensation gain, is set in the read_barometer() function in sensors.cpp.
  baroAlt : Inport
  baroAirPress : Inport  Port=2
  baroGndTemp : Inport  Port=3
  Data Store Memory : DataStoreMemory  DataStoreName=EAS2TAS  ReadBeforeWriteMsg=warning  WriteAfterWriteMsg=warning  WriteAfterReadMsg=warning  ShowAdditionalParam=off  OutDataTypeStr=single
  Data Store Memory1 : DataStoreMemory  DataStoreName=last_alt_EAS2TAS  ReadBeforeWriteMsg=warning  WriteAfterWriteMsg=warning  WriteAfterReadMsg=warning  ShowAdditionalParam=off  OutDataTypeStr=single
  Get air density ratio : MATLAB Function  TreatAsAtomicUnit=on
  Get equivalent to true airspeed EAS2TAS : MATLAB Function  TreatAsAtomicUnit=on  SystemSampleTime=simIn.param.dt
  airDensityRatio : Outport
  wires:
  Get equivalent to true airspeed EAS2TAS/1(eas2tas) -> Get air density ratio/1(eas2tas)
  Get air density ratio/1(airDensityRatio) -> airDensityRatio/1
  baroAlt/1 -> Get equivalent to true airspeed EAS2TAS/1(alt)
  baroAirPress/1 -> Get equivalent to true airspeed EAS2TAS/2(airPress)
  baroGndTemp/1 -> Get equivalent to true airspeed EAS2TAS/3(gndTemp)

== system arducopter/Throttle/Throttle Calculations/Boost and Premixing ==
  note: Angular boost and premixing.
  note: This function adds the angular boost to the desired throttle (if enabled) and outputs the maximum value between the desired throttle and the throttle, that results from mixing the desired throttle with the hover throttle.
      | (set_throttle_out() function in AC_AttitudeControl_Multi.cpp)
      | It is either called from the flightmode->run() function, if the flightmode does not include position control, or from the update_z_controller() function in AC_PosControl.cpp if position control is used.
  thrRPYMix : Inport
  thrIn : Inport  Port=2
  thrHover : Inport  Port=3
  angBst : Inport  Port=4
  Constant9 : Constant  Value=simIn.param.ATC.ANGLE_BOOST
  Throttle_In Handling : MATLAB Function  TreatAsAtomicUnit=on
  thrOutRaw : Outport
  thrAvgMax : Outport  Port=2
  wires:
  Constant9/1 -> Throttle_In Handling/4(angBstEna)
  Throttle_In Handling/2(thrAvgMax) -> thrAvgMax/1
  thrIn/1 -> Throttle_In Handling/1(thrTar)
  angBst/1 -> Throttle_In Handling/2(angBst)
  thrRPYMix/1 -> Throttle_In Handling/5(thrRpyMix)
  thrHover/1 -> Throttle_In Handling/3(thrHover)
  Throttle_In Handling/1(thrOut) -> thrOutRaw/1  "thrOutRaw"

== system arducopter/Throttle/Throttle Calculations/Lowpass Filter ==
  note: Lowpass filter throttle
      | This lowpass filter for the throttle is called in AP_MotorsMulticopter::update_throttle_filter() (AP_MotorsMulticoopter.cpp), which
      | is called in AP_MotorsMulticopter::output(), which is in turn called from Copter::motors_output in motors.cpp.
  thrOutRaw : Inport
  Constant7 : Constant  Value=simIn.param.LOOP_RATE
  Constant8 : Constant  Value=simIn.param.ATC.THR_FILT_CUTOFF
  Lowpass Filter with reset : MATLAB Function  TreatAsAtomicUnit=on
  Unit Delay1 : UnitDelay  InitialCondition=simIn.init.CTUN.ThrOut  SampleTime=-1  HasFrameUpgradeWarning=on
  thrOutFilt : Outport
  wires:
  Constant8/1 -> Lowpass Filter with reset/2(cutoff_freq)
  Constant7/1 -> Lowpass Filter with reset/3(loop_rate)
  Unit Delay1/1 -> Lowpass Filter with reset/4(lastSamp)
  thrOutRaw/1 -> Lowpass Filter with reset/1(in)
  Lowpass Filter with reset/1(out) -> thrOutFilt/1, Unit Delay1/1  "thrOutFilt"

== system arducopter/Throttle/Throttle Calculations/Throttle Hover ==
  note: Update throttle hover
  note: The parameters THST_HOVER_TC, THST_HOVER_MIN and THST_HOVER_MAX are defined in AP_MotorsMulticopter.h. The value 0.01 for dt is taken from the function call Copter::update_throttle_hover() in Attitude.cpp.
      | The parameters THST_HOVER and HOVER_LEARN are defined in AP_MotorsMulticopter.cpp. They are set in the initialization of the copter with the parameters MOT_THST_HOVER and MOT_THST_LEARN
      | respectively.
  note: Subsystem for updating throttle hover. Runs as a atomic unit with a sample time of 10 ms (100 Hz) since the scheduler task for updating the throttle hover value is called with this frequency (see Copter.cpp, SCHED_TASK(update_throttle_hover, 100, 90) ).
      | Simply uses the default hover value, when manual throttle is active (as the first condition) or thr_hover_learn is not activated (as the secondary condition).
  zVelAct : Inport
  zVelDes : Inport  Port=2
  thrAct : Inport  Port=3
  Constant : Constant  Value=0.01  OutDataTypeStr=single
  Constant1 : Constant  Value=simIn.param.MOT.THST_HOVER_MAX
  Constant2 : Constant  Value=simIn.param.MOT.THST_HOVER_MIN
  Constant3 : Constant  Value=simIn.param.MOT.THST_HOVER_TC
  Constant4 : Constant  Value=simIn.param.MOT.THST_HOVER
  Constant5 : Constant  Value=simIn.param.MOT.HOVER_LEARN
  Constant6 : Constant  Value=simIn.param.MODE.THR_MAN_FLG
  Data Store Memory : DataStoreMemory  DataStoreName=thrHoverAct  ReadBeforeWriteMsg=warning  WriteAfterWriteMsg=warning  WriteAfterReadMsg=warning  InitialValue=simIn.init.CTUN.ThrHov  ShowAdditionalParam=off  OutDataTypeStr=single
  Throttle Hover Calculation : MATLAB Function  TreatAsAtomicUnit=on
  thrHover : Outport
  wires:
  Throttle Hover Calculation/1(thrHover) -> thrHover/1  "thrHover"
  Constant/1 -> Throttle Hover Calculation/1(dt)
  thrAct/1 -> Throttle Hover Calculation/2(thrAct)
  Constant1/1 -> Throttle Hover Calculation/5(thstHoverMax)
  Constant2/1 -> Throttle Hover Calculation/6(thstHoverMin)
  Constant3/1 -> Throttle Hover Calculation/7(thstHoverTC)
  Constant4/1 -> Throttle Hover Calculation/8(thstHoverDefault)
  Constant5/1 -> Throttle Hover Calculation/9(hoverLearn)
  Constant6/1 -> Throttle Hover Calculation/10(thrMan)
  zVelAct/1 -> Throttle Hover Calculation/4(zVelAct)
  zVelDes/1 -> Throttle Hover Calculation/3(zVelDes)

== system arducopter/Throttle/Throttle Calculations/Throttle Limiting based on battery state ==
  note: thr_limit and thr_thst_max are set to 1.0 as initial value, since both values are set to 1.0
      | when the motors are disarmed (see get_current_limit_max_throttle()), which
      | means both quantities are always set to 1.0 at the beginning of a flight.
  note: Calculates the throttle limit that represents the maximum additional throttle on top of the hover throttle based on the ratio between actual and maximum battery current. The higher the ratio (and the higher the utilization repectively), the lower the throttle limit. The acutal current is taken as minimum for the limit.
  note: Calculates maximum lift "lift_max" based on resting battery voltage (battery voltage reduced by sag that results from internal resistance, calculated in AP_BattMonitor_Backend.cpp, update_resistance_estimate()) and sets a new lower limit for the voltage "bat_volt_min" below that no additional scaling of thrust is conducted.
  note: Calculation of quantities to limit or scale thrust output.
  batRestVoltEst : Inport
  batCurr : Inport  Port=2
  batRes : Inport  Port=3
  batVolt : Inport  Port=4
  thrHover : Inport  Port=5
  Constant11 : Constant  Value=simIn.param.LOOP_RATE
  Constant12 : Constant  Value=simIn.param.MOT.THST_EXPO
  Constant13 : Constant  Value=simIn.param.MOT.BAT_VOLT_MIN
  Constant14 : Constant  Value=simIn.param.MOT.BAT_VOLT_MAX
  Constant15 : Constant  Value=simIn.param.LOOP_RATE
  Constant16 : Constant  Value=simIn.param.MOT.BAT_CURR_MAX
  Constant17 : Constant  Value=simIn.param.MOT.BAT_CURR_TC
  Get current throttle limit : MATLAB Function  TreatAsAtomicUnit=on
  IC : InitialCondition
  Unit Delay3 : UnitDelay  InitialCondition=simIn.init.BAT.RestVoltEst/simIn.param.MOT.BAT_VOLT_MIN  SampleTime=-1  HasFrameUpgradeWarning=on
  Unit Delay4 : UnitDelay  InitialCondition=1.0  SampleTime=-1  HasFrameUpgradeWarning=on
  Update Lift Max from Battery Voltage : MATLAB Function  TreatAsAtomicUnit=on
  liftMax : Outport
  batVoltRestEstAct : Outport  Port=2
  thrThstMax : Outport  Port=3
  wires:
  Unit Delay3/1 -> Update Lift Max from Battery Voltage/1(battVoltFiltLast)
  Constant16/1 -> Get current throttle limit/2(batCurrMax)
  Constant17/1 -> Get current throttle limit/3(batCurrT)
  batVolt/1 -> Get current throttle limit/7(batVolt)
  Update Lift Max from Battery Voltage/1(battVoltFilt) -> Unit Delay3/1
  Constant14/1 -> Update Lift Max from Battery Voltage/3(battVoltMax)
  thrHover/1 -> Get current throttle limit/8(thrHover)
  Constant13/1 -> Update Lift Max from Battery Voltage/4(battVoltMin)
  Update Lift Max from Battery Voltage/3(battVoltMinAct) -> Get current throttle limit/1(batVoltMin)
  batRestVoltEst/1 -> Update Lift Max from Battery Voltage/2(battVoltRestEst)
  Update Lift Max from Battery Voltage/2(liftMax) -> liftMax/1
  batCurr/1 -> Get current throttle limit/5(batCurr)
  Constant12/1 -> Update Lift Max from Battery Voltage/5(thstCurveExpo)
  Constant15/1 -> Get current throttle limit/4(loop_rate)
  Unit Delay4/1 -> Get current throttle limit/9(thrLimitLast)
  batRes/1 -> Get current throttle limit/6(batRes)
  Get current throttle limit/2(thrLimit) -> Unit Delay4/1  "thrLimit"
  Constant11/1 -> Update Lift Max from Battery Voltage/6(loop_rate)
  Get current throttle limit/1(thrThstMax) -> IC/1
  Update Lift Max from Battery Voltage/4(battVoltRestEstAct) -> batVoltRestEstAct/1
  IC/1 -> thrThstMax/1
